simulink model "ssc_hydromech_power_split_cvt_engine"  (R2025a)
settings: Solver=VariableStepAuto  StartTime=0.0  StopTime=70  RelTol=1e-3
StartFcn:
  | tic
StopFcn:
  | Elapsed_Sim_Time = toc;
  | disp(['Elapsed Sim Time = ' num2str(Elapsed_Sim_Time)]);
undefined symbols (not defined in the file or in its folder): HMPST
libraries: sm_wheel_loader_lib x9, fl_lib x4, sdl_lib x2, simulink x1, nesl_utility x1
Description:
  | Hydromechanical Power Split CVT with Engine
  | Copyright 2023-2025 The MathWorks, Inc.
settings Model: TunableVars=Init_Veh_TopSpeed  TunableVarsStorageClass=Auto  Creator=Shusen Zhang  LastModifiedBy=smiller
settings SolverCC: MaxConsecutiveMinStep=5
settings DataIOCC: ReturnWorkspaceOutputs=off  SignalLoggingName=logsout_ssc_hydromech_power_split_cvt_engine
settings DebuggingCC: UnderspecifiedInitializationDetection=Classic  MergeDetectMultiDrivingBlocksExec=none
settings ModelReferenceCC: PropagateSignalLabelsOutOfModel=off
settings RTWCC: GPUComputeCapability=3.5
settings SimscapeCC: SimscapeLogType=all  SimscapeLogName=simlog_ssc_hydromech_power_split_cvt_engine  SimscapeLogLimitData=off
settings ExplorerConfigSet: SimMechanicsOpenEditorOnUpdate=off

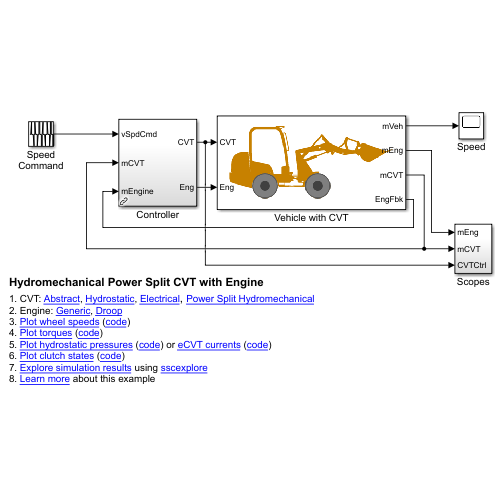
[thumbnail: Simulink's stored preview of the top-level diagram]
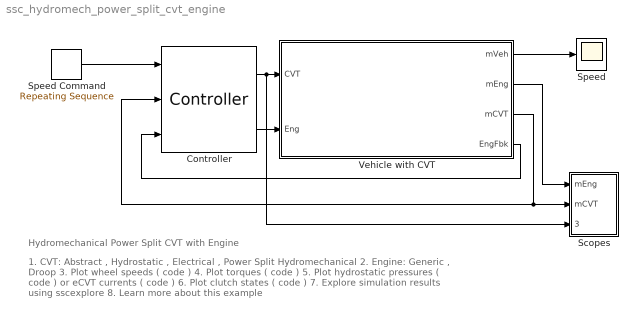
== system ssc_hydromech_power_split_cvt_engine ==
  note: Hydromechanical Power Split CVT with Engine
  note: 1. CVT: Abstract , Hydrostatic , Electrical , Power Split Hydromechanical
      | 2. Engine: Generic , Droop
      | 3. Plot wheel speeds ( code )
      | 4. Plot torques ( code )
      | 5. Plot hydrostatic pressures ( code ) or eCVT currents ( code )
      | 6. Plot clutch states ( code )
      | 7. Explore simulation results using sscexplore
      | 8. Learn more about this example
  Controller : sm_wheel_loader_lib/Controller  SystemSampleTime=-1  VariantActivationTime=update diagram  EmptyChoice=off  PassThrough=off  PassThroughVariantControl=(default)  EmptyChoiceVariantControl=(default)  AllowFlexibleInterface=on  Latency=0  AutoFrameSizeCalculation=off
  Scopes : Subsystem
  Speed : Scope
      settings: ActiveDisplayYMinimum=-9.37204  ActiveDisplayYMaximum=9.37302
  Speed Command : simulink/Sources/Repeating Sequence  rep_seq_t=[0 10 12 15 17 32 34 37 39 41 43 46 48 63 65 68 70]  rep_seq_y=[0 0 1 1 0 0 -1 -1 0 0 1 1 0 0 -1 -1 0]*25
  Vehicle with CVT : Subsystem
      mask Display: image('sm_wheel_loader_vehicle1D_IMAGE.png');
  wires:
  Controller/1 -> Scopes/3(CVTCtrl), Vehicle with CVT/1(CVT)
  Controller/2 -> Vehicle with CVT/2(Eng)
  Vehicle with CVT/3(mCVT) -> Scopes/2(mCVT), Controller/2
  Vehicle with CVT/4(EngFbk) -> Controller/3
  Speed Command/1 -> Controller/1
  Vehicle with CVT/2(mEng) -> Scopes/1(mEng)
  Vehicle with CVT/1(mVeh) -> Speed/1

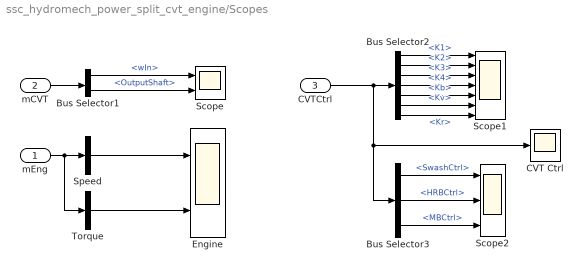
== system ssc_hydromech_power_split_cvt_engine/Scopes ==
  mEng : Inport
  mCVT : Inport  Port=2
  CVTCtrl : Inport  Port=3
  Bus Selector1 : BusSelector  OutputSignals=wIn,OutputShaft
  Bus Selector2 : BusSelector  OutputSignals=K1,K2,K3,K4,Kb,Kv,Kr
  Bus Selector3 : BusSelector  OutputSignals=SwashCtrl,HRBCtrl,MBCtrl
  CVT Ctrl : Scope
      settings: ActiveDisplayYMinimum=-0.96987  ActiveDisplayYMaximum=1.21887  DataLoggingVariableName=ScopeData2
  Engine : Scope  NumInputPorts=2
      settings: ActiveDisplayYMinimum=-286.4333  ActiveDisplayYMaximum=2577.89969
  Scope : Scope  NumInputPorts=2
      settings: ActiveDisplayYMinimum=-1460.02488  ActiveDisplayYMaximum=1460.04785  DataLoggingVariableName=ScopeData4
  Scope1 : Scope  NumInputPorts=7
      settings: ActiveDisplayYMinimum=-0.125  ActiveDisplayYMaximum=1.125  DataLoggingVariableName=ScopeData3
  Scope2 : Scope  NumInputPorts=3
      settings: ActiveDisplayYMinimum=-0.96987  ActiveDisplayYMaximum=1.21887  DataLoggingVariableName=ScopeData4
  Speed : BusSelector  OutputSignals=w.cmd,w.meas  OutputAsBus=on
  Torque : BusSelector  OutputSignals=trq.Cmd  OutputAsBus=on
  wires:
  Bus Selector1/1 -> Scope/1  "<wIn>"
  Bus Selector1/2 -> Scope/2  "<OutputShaft>"
  mCVT/1 -> Bus Selector1/1
  Bus Selector2/1 -> Scope1/1  "<K1>"
  CVTCtrl/1 -> Bus Selector3/1, CVT Ctrl/1, Bus Selector2/1
  Bus Selector3/2 -> Scope2/2  "<HRBCtrl>"
  Bus Selector2/3 -> Scope1/3  "<K3>"
  Bus Selector2/6 -> Scope1/6  "<Kv>"
  Bus Selector2/2 -> Scope1/2  "<K2>"
  Bus Selector3/1 -> Scope2/1  "<SwashCtrl>"
  Bus Selector3/3 -> Scope2/3  "<MBCtrl>"
  Bus Selector2/4 -> Scope1/4  "<K4>"
  Bus Selector2/5 -> Scope1/5  "<Kb>"
  Bus Selector2/7 -> Scope1/7  "<Kr>"
  mEng/1 -> Torque/1, Speed/1
  Torque/1 -> Engine/2
  Speed/1 -> Engine/1

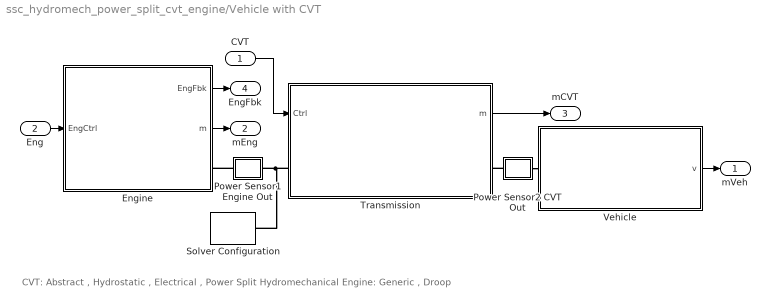
== system ssc_hydromech_power_split_cvt_engine/Vehicle with CVT ==
  note: CVT: Abstract , Hydrostatic , Electrical , Power Split Hydromechanical
      | Engine: Generic , Droop
  CVT : Inport
  Eng : Inport  Port=2
  Engine : Subsystem  Variant=on  VariantControlMode=label  VariantControl=Choice  LabelModeActiveChoice=Droop
      settings: AttributesFormatString=%<LabelModeActiveChoice>
  Power Sensor1 Engine Out : Subsystem
  Power Sensor2 CVT Out : Subsystem
  Solver Configuration : nesl_utility/Solver Configuration  PhysicalDomain=network_engine_domain  SubClassName=solver  LeftPortType=input  RightPortType=generic  Tones=[]  Harmonics=[]  SimulateNoise=off  Profile=off  UseLocalSampling=off  EnableSwitchedLinearOptims=on  FrequencyDomain=off  UseCCode=off  RelTol=0.001  AbsTol=1e-06  MinStep=1e-09  ToWorkspace=off  RevertToSquareIcSolve=off  NumHomotopyIterations=100  PhasorMode=off  PhasorModeNumHarmonics=1  ConsistencySolver=NEWTON_XTOL_AFTER_FTOL  IndexReductionMethod=DerivativeReplacement  DoDC=off  ResidualTolerance=1e-09  ConsistencyTolSource=GLOBAL  ConsistencyAbsTol=0.001  ConsistencyRelTol=0.001  ConsistencyTolFactor=0.001  UseLocalSolver=off  LocalSolverChoice=NE_BACKWARD_EULER_ADVANCER  ResolveIndetEquations=on  FunctionEvalNumThread=1  LocalSolverSampleTime=0.001  DoFixedCost=off  MaxNonlinIter=1  MaxModeIter=2  ComputeImpulses=off  ImpulseIterations=2  LinearAlgebra=Sparse  LinearAlgebraNumThread=0  EquationFormulation=NE_TIME_EF  DelaysMemoryBudget=1024  AutomaticFiltering=on  FilteringTimeConstant=0.001  PartitionStorageMethod=AS_NEEDED  PartitionMemoryBudget=1024  PartitionMethod=FAST  MultibodyUseLocalSolver=off  MultibodyLocalSolverChoice=ODE1  MultibodyLocalSolverSampleTime=0.001
  Transmission : Subsystem  Variant=on  VariantControlMode=label  VariantControl=Choice  LabelModeActiveChoice=Abstract
      settings: AttributesFormatString=%<LabelModeActiveChoice>
  Vehicle : Subsystem
      mask Display: image('sm_wheel_loader_vehicle1D_IMAGE.png');
  mVeh : Outport
  mEng : Outport  Port=2
  mCVT : Outport  Port=3
  EngFbk : Outport  Port=4
  wires:
  CVT/1 -> Transmission/1(Ctrl)
  Transmission/1(m) -> mCVT/1
  Eng/1 -> Engine/1(EngCtrl)
  Engine/1(EngFbk) -> EngFbk/1
  Engine/2(m) -> mEng/1
  Vehicle/1(v) -> mVeh/1
  connections:
  Power Sensor2 CVT Out/RConn1 -- Vehicle/LConn1
  Transmission/LConn1 -- Solver Configuration/RConn1 -- Power Sensor1 Engine Out/RConn1
  Power Sensor1 Engine Out/LConn1 -- Engine/RConn1
  Power Sensor2 CVT Out/LConn1 -- Transmission/RConn1

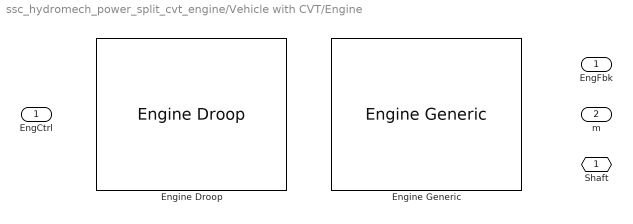
== system ssc_hydromech_power_split_cvt_engine/Vehicle with CVT/Engine ==
  EngCtrl : Inport
  Engine Droop : sm_wheel_loader_lib/Engine Droop  SystemSampleTime=-1  VariantControl=Droop  VariantActivationTime=update diagram  EmptyChoice=off  PassThrough=off  PassThroughVariantControl=(default)  EmptyChoiceVariantControl=(default)  AllowFlexibleInterface=on  Latency=0  AutoFrameSizeCalculation=off
  Engine Generic : sm_wheel_loader_lib/Engine Generic  SystemSampleTime=-1  VariantControl=Generic  VariantActivationTime=update diagram  EmptyChoice=off  PassThrough=off  PassThroughVariantControl=(default)  EmptyChoiceVariantControl=(default)  AllowFlexibleInterface=on  Latency=0  AutoFrameSizeCalculation=off
  Shaft : PMIOPort  Side=Right
  EngFbk : Outport
  m : Outport  Port=2

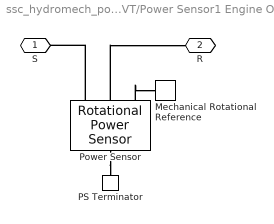
== system ssc_hydromech_power_split_cvt_engine/Vehicle with CVT/Power Sensor1 Engine Out ==
  Mechanical Rotational Reference : fl_lib/Mechanical/Rotational Elements/Mechanical Rotational Reference
  PS Terminator : fl_lib/Physical Signals/Sinks/PS Terminator
  Power Sensor : sdl_lib/Sensors/Rotational Power Sensor  measurement_type=sdl.enum.rotationalPowerSensorType.instantaneous  averaging_period=1 s  max_frequency=1000 Hz  max_speed=1000 rpm
      settings: InternalSimscapePortConfiguration="{\"Bottom\":[],\"Left\":[{\"id\":\"S\",\"label\":\"S\",\"type\":\"foundation.mechanical.rotational.rotational\"},{\"id\":\"R\",\"label\":\"R\",\"type\":\"foundation.mechanical.rotational.rotational\"},{\"id\":\"C\",\"label\":\"C\",\"type\":\"foundation.mechanical.rotational.rotational\"}],\"Right\":[{\"id\":\"P\",\"label\":\"P\",\"type\":\"output\"}],\"Top\":[]}"
  S : PMIOPort  Side=Left
  R : PMIOPort  Port=2  Side=Right
  connections:
  Power Sensor/RConn1 -- PS Terminator/LConn1
  Power Sensor/LConn3 -- Mechanical Rotational Reference/LConn1
  Power Sensor/LConn2 -- R/RConn1
  Power Sensor/LConn1 -- S/RConn1

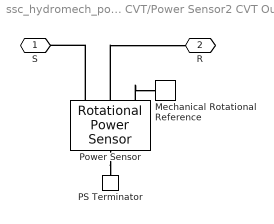
== system ssc_hydromech_power_split_cvt_engine/Vehicle with CVT/Power Sensor2 CVT Out ==
  Mechanical Rotational Reference : fl_lib/Mechanical/Rotational Elements/Mechanical Rotational Reference
  PS Terminator : fl_lib/Physical Signals/Sinks/PS Terminator
  Power Sensor : sdl_lib/Sensors/Rotational Power Sensor  measurement_type=sdl.enum.rotationalPowerSensorType.instantaneous  averaging_period=1 s  max_frequency=1000 Hz  max_speed=1000 rpm
      settings: InternalSimscapePortConfiguration="{\"Bottom\":[],\"Left\":[{\"id\":\"S\",\"label\":\"S\",\"type\":\"foundation.mechanical.rotational.rotational\"},{\"id\":\"R\",\"label\":\"R\",\"type\":\"foundation.mechanical.rotational.rotational\"},{\"id\":\"C\",\"label\":\"C\",\"type\":\"foundation.mechanical.rotational.rotational\"}],\"Right\":[{\"id\":\"P\",\"label\":\"P\",\"type\":\"output\"}],\"Top\":[]}"
  S : PMIOPort  Side=Left
  R : PMIOPort  Port=2  Side=Right
  connections:
  Power Sensor/LConn1 -- S/RConn1
  Power Sensor/LConn2 -- R/RConn1
  Power Sensor/LConn3 -- Mechanical Rotational Reference/LConn1
  Power Sensor/RConn1 -- PS Terminator/LConn1

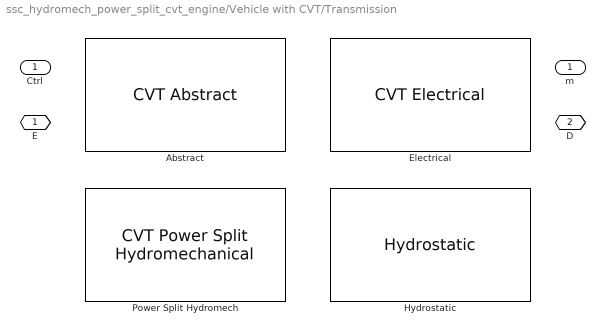
== system ssc_hydromech_power_split_cvt_engine/Vehicle with CVT/Transmission ==
  Ctrl : Inport
  Abstract : sm_wheel_loader_lib/CVT Abstract  VariantControl=Abstract  dShaftE=HMPST.AbstractCVT.dInput  dShaftD=HMPST.AbstractCVT.dOutput  k=HMPST.AbstractCVT.kCompliance  d=HMPST.AbstractCVT.dCompliance
  Electrical : sm_wheel_loader_lib/CVT Electrical  VariantControl=Electrical
  Hydrostatic : sm_wheel_loader_lib/Hydrostatic  SystemSampleTime=-1  VariantControl=Hydrostatic  VariantActivationTime=update diagram  EmptyChoice=off  PassThrough=off  PassThroughVariantControl=(default)  EmptyChoiceVariantControl=(default)  AllowFlexibleInterface=on  Latency=0  AutoFrameSizeCalculation=off
  Power Split Hydromech : sm_wheel_loader_lib/CVT Power Split Hydromechanical  SystemSampleTime=-1  VariantControl=Power_Split_HM  VariantActivationTime=update diagram  EmptyChoice=off  PassThrough=off  PassThroughVariantControl=(default)  EmptyChoiceVariantControl=(default)  AllowFlexibleInterface=on  Latency=0  AutoFrameSizeCalculation=off
      settings: LibrarySourceBlock=sm_wheel_loader_lib/CVT Powersplit Hydromechanical
  E : PMIOPort  Side=Left
  D : PMIOPort  Port=2  Side=Right
  m : Outport

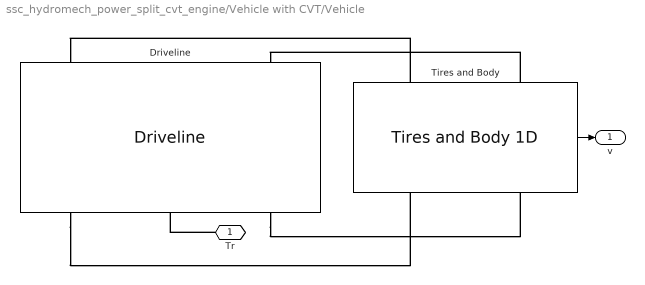
== system ssc_hydromech_power_split_cvt_engine/Vehicle with CVT/Vehicle ==
  Driveline : sm_wheel_loader_lib/Wheel Loader Vehicle/Driveline/Driveline/Driveline 1D/Driveline  SystemSampleTime=-1  VariantActivationTime=update diagram  EmptyChoice=off  PassThrough=off  PassThroughVariantControl=(default)  EmptyChoiceVariantControl=(default)  AllowFlexibleInterface=on  Latency=0  AutoFrameSizeCalculation=off
  Tires and Body : sm_wheel_loader_lib/Tires and Body 1D  SystemSampleTime=-1  VariantActivationTime=update diagram  EmptyChoice=off  PassThrough=off  PassThroughVariantControl=(default)  EmptyChoiceVariantControl=(default)  AllowFlexibleInterface=on  Latency=0  AutoFrameSizeCalculation=off
      settings: PortSchema="{\"entries\":[{\"content\":{\"sides\":[{\"content\":{\"connectorIds\":[\"LConn1\",\"LConn2\"]},\"type\":\"ConnectorPlacement.EquallySpacedRectSide\",\"uuid\":\"f6e4eca3-fb02-4523-87a7-c8328825f67f\"},{\"content\":{\"connectorIds\":[\"RConn1\",\"RConn2\"],\"side\":\"RIGHT\"},\"type\":\"ConnectorPlacement.EquallySpacedRectSide\",\"uuid\":\"a01e7d42-3992-448e-add1-f2755d8f064c\"},{\"content\":{\"connectorIds\":[\"Out1\"],\"side\":\"TOP\"},\"type\":\"ConnectorPlacement.EquallySpacedRectSide\",\"uuid\":\"cf483cf6-51ef-4c82-b2ec-fd42745a5c51\"},{\"content\":{\"side\":\"BOTTOM\"},\"type\":\"ConnectorPlacement.EquallySpacedRectSide\",\"uuid\":\"9bbb772c-3b9f-4e30-8c40-373d820ff5eb\"}]},\"type\":\"ConnectorPlacement.EquallySpacedConnector\",\"uuid\":\"52398d34-f462-4e1c-abff-1dda3b221c82\"}],\"packageUris\":[\"http://schema.mathworks.com/mf0/Connector/R2020b\"],\"version\":\"1.0\"}"
  Tr : PMIOPort  Side=Left
  v : Outport
  wires:
  Tires and Body/1 -> v/1
  connections:
  Tires and Body/LConn1 -- Driveline/LConn3
  Tires and Body/LConn2 -- Driveline/LConn1
  Driveline/RConn3 -- Tires and Body/RConn1
  Driveline/RConn1 -- Tires and Body/RConn2
  Tr/RConn1 -- Driveline/RConn2
